simulink model "PendulumQuickStart_RL"  (R2025a)
settings: Solver=ode4  StartTime=0.0  StopTime=inf  FixedStep=0.004  RelTol=1e-3  EnableMultiTasking=on
InitFcn:
  | LoadCalibrateData
  | Linear_System_Model_LQR_Matrixes
values from neighbouring files (symbols this model uses):
  Beq = 30.0    (= 30)    [lqrs13s17_sim.m]
  K = 2/DT    [ol_center_sim.m]
  Kb = 0.11693    [lqrs13s17_sim.m]
  Kt = 0.08505    [lqrs13s17_sim.m]
  Mc = 0.4719    [ol_center_sim.m]
  Mp = 0.1679    [ol_center_sim.m]
  Rm = 2.12    [lqrs13s17_sim.m]
  rmp = 0.013745    [lqrs13s17_sim.m]
undefined symbols (not defined in the file or in its folder): Nbar
libraries: raspberrypiCommlib x2, simulink x1
settings Model: SimulationMode=external  ExtModeTrigDuration=2  Creator=Mustafa  LastModifiedBy=chenyihong
settings SolverCC: ExtrapolationOrder=2.0  AlgebraicLoopSolver=TrustRegion  PositivePriorityOrder=on  AutoInsertRateTranBlk=on
settings DataIOCC: ReturnWorkspaceOutputs=off
settings OptimizationCC: PassReuseOutputArgsAs=Individual arguments  MaxStackSize=200000  EfficientTunableParamExpr=on
settings DebuggingCC: ParameterTunabilityLossMsg=error  UnconnectedInputMsg=warning  UnconnectedOutputMsg=warning  UnconnectedLineMsg=warning  ArithmeticOperatorsInVariantConditions=warning
settings HardwareCC: ProdBitPerLong=64.0  ProdLargestAtomicInteger=LongLong  ProdLargestAtomicFloat=Double  ProdLongLongMode=on  ProdHWDeviceType=ARM Compatible->ARM Cortex-A (64-bit)
settings ModelReferenceCC: EnableRefExpFcnMdlSchedulingChecks=on
settings SFSimCC: SimUseLocalCustomCode=off  CustomCodeUndefinedFunction=UseInterfaceOnly
settings RTWCC: SystemTargetFile=ert.tlc  HardwareBoard=Raspberry Pi (64bit)  TLCOptions="-aInlineSetEventsForThisBaseRateFcn=TLC_FALSE -aSuppressMultiTaskScheduler=TLC_FALSE  -aRateBasedStepFcn=0"  TemplateMakefile=ert_default_tmf  GenerateReport=on  RTWUseLocalCustomCode=off  Toolchain=GNU GCC Embedded Linux  BuildConfiguration=Faster Runs  IncludeHyperlinkInReport=on  LaunchReport=on  GenerateTraceInfo=on  GenerateTraceReport=on  GenerateTraceReportSl=on  GenerateTraceReportSf=on  GenerateTraceReportEml=on  GPUComputeCapability=3.5  DLArmComputeVersion=19.05  Description=Embedded Coder
settings CodeAppCC: ForceParamTrailComments=on  IgnoreCustomStorageClasses=off  OperatorAnnotations=on  SimulinkDataObjDesc=on  SFDataObjDesc=on  InsertBlockDesc=on
settings ERTTargetCC: ExtMode=on  ExtModeTransport=2.0  ExtModeMexArgs='127.0.0.1' 0 17725  InlinedParameterPlacement=Hierarchical  DynamicArrayContainerType=coder::array  CodeReplacementLibrary=ARM Cortex-A CMSIS  SupportContinuousTime=on  SupportVariableSizeSignals=on
settings SimscapeCC: SimscapeLogDecimation=1  SimscapeLogDataHistory=5000

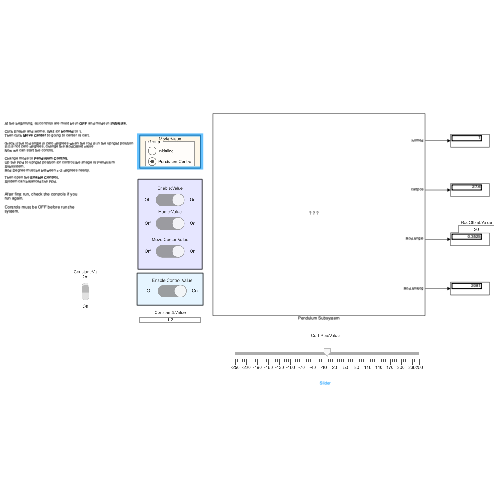
[thumbnail: Simulink's stored preview of the top-level diagram]
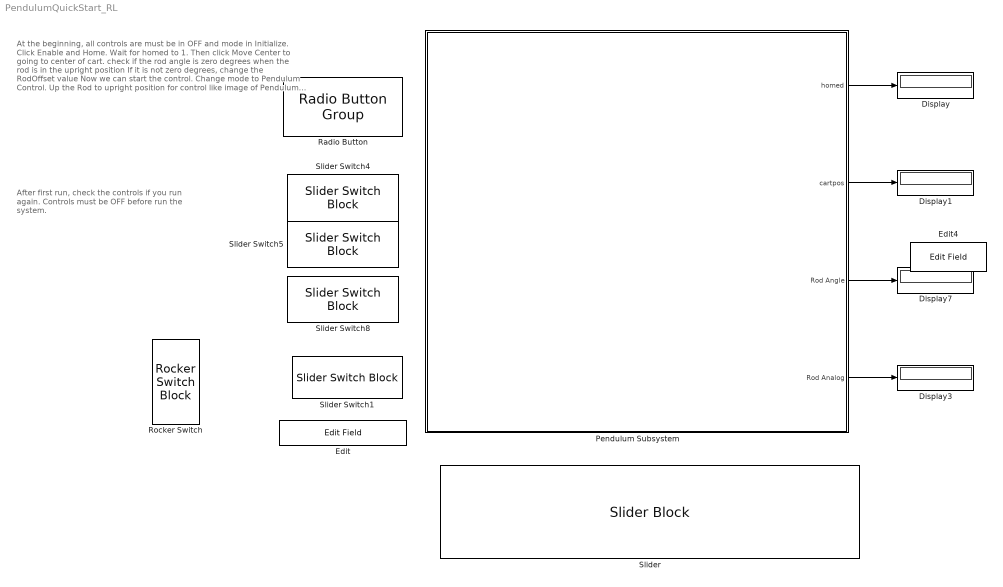
== system PendulumQuickStart_RL ==
  note: At the beginning, all controls are must be in OFF and mode in Initialize.
      |
      | Click Enable and Home. Wait for homed to 1.
      | Then click Move Center to going to center of cart.
      |
      | check if the rod angle is zero degrees when the rod is in the upright position
      | If it is not zero degrees, change the RodOffset value
      | Now we can start the control.
      |
      | Change mode to Pendulum Control.
      | Up the Rod to upright position for control like image of Pendulum Subsystem.
      | Rod Degree must be between +-2 degrees nearly.
      |
      | Then open the Enable Control.
      | System can balanced the Rod.
  note: After first run, check the controls if you run again.
      |
      | Controls must be OFF before run the system.
  Display{,1,3,7} (4 alike) : Display
  Edit : EditField  ShowInitialText=on  Alignment=Center
  Edit4 : EditField  Alignment=Center
  Pendulum Subsystem : Subsystem
      mask Display: image('Resim1.png'); % Use "Edit Image" on toolstrip to change.
  Radio Button : RadioButtonGroup  SelectedLabel=Pendulum Control  ButtonGroupName=Group
  Rocker Switch : RockerSwitchBlock
  Slider : SliderBlock  ScaleMin=-250  ScaleMax=250
  Slider Switch{1,4..5,8} (4 alike) : SliderSwitchBlock
  wires:
  Pendulum Subsystem/1(homed) -> Display/1
  Pendulum Subsystem/2(cartpos) -> Display1/1
  Pendulum Subsystem/3(Rod Angle) -> Display7/1
  Pendulum Subsystem/4(Rod Analog) -> Display3/1

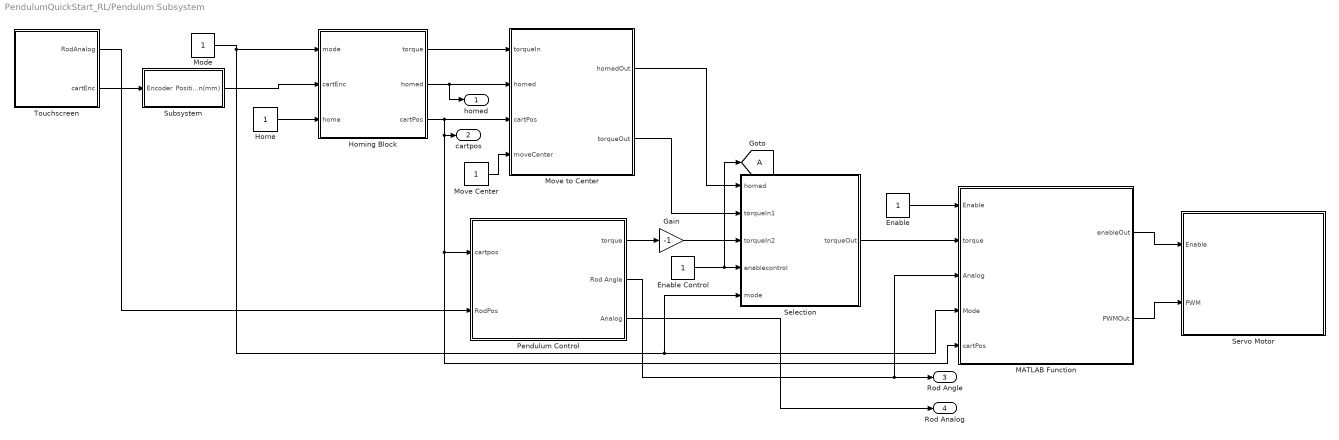
== system PendulumQuickStart_RL/Pendulum Subsystem ==
  Enable : Constant
  Enable Control : Constant
  Gain : Gain  Gain=-1
  Goto : Goto  TagVisibility=global
  Home : Constant
  Homing Block : MATLAB Function  TreatAsAtomicUnit=on
  MATLAB Function : MATLAB Function  TreatAsAtomicUnit=on
  Mode : Constant
  Move Center : Constant
  Move to Center : MATLAB Function  TreatAsAtomicUnit=on
  Pendulum Control : Subsystem
  Selection : MATLAB Function  TreatAsAtomicUnit=on
  Servo Motor : Subsystem
  Subsystem : Subsystem
  Touchscreen : Subsystem
  homed : Outport
  cartpos : Outport  Port=2
  Rod Angle : Outport  Port=3
  Rod Analog : Outport  Port=4
  wires:
  Mode/1 -> Selection/5(mode), MATLAB Function/4(Mode), Homing Block/1(mode)
  Homing Block/2(homed) -> homed/1, Move to Center/2(homed)
  Home/1 -> Homing Block/3(home)
  Move Center/1 -> Move to Center/4(moveCenter)
  Pendulum Control/1(torque) -> Gain/1
  Homing Block/1(torque) -> Move to Center/1(torqueIn)
  Move to Center/1(homedOut) -> Selection/1(homed)
  Move to Center/2(torqueOut) -> Selection/2(torqueIn1)
  Selection/1(torqueOut) -> MATLAB Function/2(torque)
  Enable Control/1 -> Goto/1, Selection/4(enablecontrol)
  MATLAB Function/1(enableOut) -> Servo Motor/1(Enable)
  Pendulum Control/2(Rod Angle) -> MATLAB Function/3(Analog), Rod Angle/1
  Enable/1 -> MATLAB Function/1(Enable)
  Touchscreen/2(cartEnc) -> Subsystem/1(Encoder)
  Subsystem/1(Position(mm)) -> Homing Block/2(cartEnc)
  Pendulum Control/3(Analog) -> Rod Analog/1
  Homing Block/3(cartPos) -> MATLAB Function/5(cartPos), Pendulum Control/1(cartpos), cartpos/1, Move to Center/3(cartPos)
  Touchscreen/1(RodAnalog) -> Pendulum Control/2(RodPos)
  MATLAB Function/2(PWMOut) -> Servo Motor/2(PWM)
  Gain/1 -> Selection/3(torqueIn2)

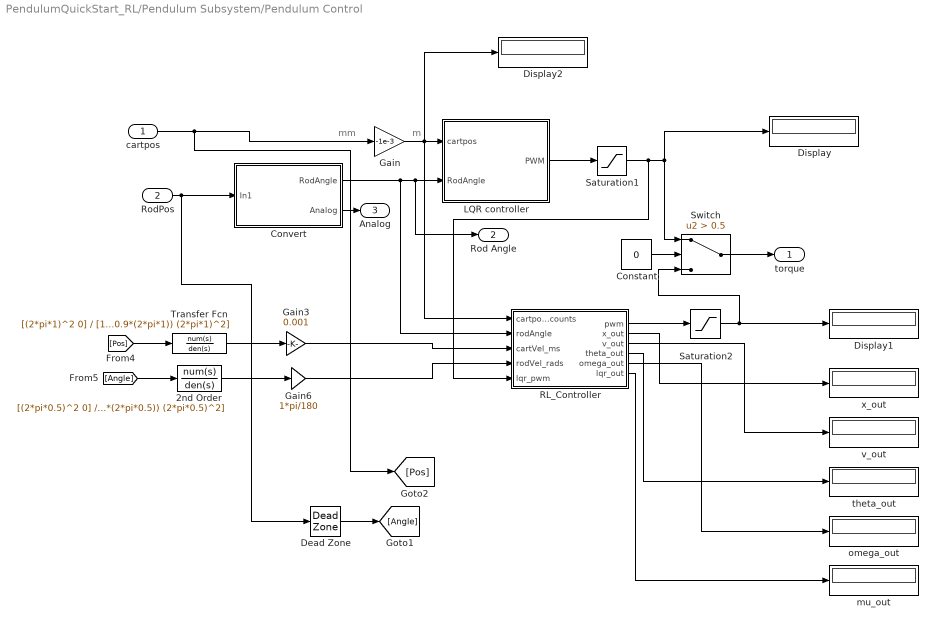
== system PendulumQuickStart_RL/Pendulum Subsystem/Pendulum Control ==
  note: m
  note: mm
  cartpos : Inport
  RodPos : Inport  Port=2
  2nd Order : TransferFcn  Numerator=[(2*pi*0.5)^2 0]  Denominator=[1 (2*0.9*(2*pi*0.5)) (2*pi*0.5)^2]
  Constant : Constant  Value=0
  Convert : Subsystem
  Dead Zone : DeadZone  LowerValue=-0.05  UpperValue=+0.05
  Display : Display
  Display1 : Display
  Display2 : Display
  Gain : Gain  Gain=-1e-3
  Gain3 : Gain  Gain=0.001
  Gain6 : Gain  Gain=1*pi/180
  LQR controller : Subsystem
  RL_Controller : MATLAB Function  TreatAsAtomicUnit=on
  Saturation1 : Saturate  UpperLimit=1000  LowerLimit=-1000
  Saturation2 : Saturate  UpperLimit=1000  LowerLimit=-1000
  Switch : Switch  Criteria=u2 > Threshold  Threshold=0.5  SaturateOnIntegerOverflow=off  InputSameDT=off
  Transfer Fcn : TransferFcn  Numerator=[(2*pi*1)^2 0]  Denominator=[1 (2*0.9*(2*pi*1)) (2*pi*1)^2]
  mu_out : Display
  omega_out : Display
  theta_out : Display
  v_out : Display
  x_out : Display
  torque : Outport
  Rod Angle : Outport  Port=2
  Analog : Outport  Port=3
  wires:
  cartpos/1 -> Gain/1, [Pos]
  Convert/2(Analog) -> Analog/1
  RodPos/1 -> Dead Zone/1, Convert/1(In1)
  Transfer Fcn/1 -> Gain3/1
  2nd Order/1 -> Gain6/1
  [Pos] -> Transfer Fcn/1
  [Angle] -> 2nd Order/1
  Saturation1/1 -> RL_Controller/5(lqr_pwm), Switch/1, Display/1
  Constant/1 -> Switch/2
  Switch/1 -> torque/1
  Dead Zone/1 -> [Angle]
  LQR controller/1(PWM) -> Saturation1/1
  Gain6/1 -> RL_Controller/4(rodVel_rads)
  RL_Controller/1(pwm) -> Saturation2/1
  Saturation2/1 -> Switch/3, Display1/1
  Gain/1 -> Display2/1, RL_Controller/1(cartpos_counts), LQR controller/1(cartpos)
  Convert/1(RodAngle) -> RL_Controller/2(rodAngle), LQR controller/2(RodAngle), Rod Angle/1
  Gain3/1 -> RL_Controller/3(cartVel_ms)
  RL_Controller/2(x_out) -> x_out/1
  RL_Controller/3(v_out) -> v_out/1
  RL_Controller/4(theta_out) -> theta_out/1
  RL_Controller/5(omega_out) -> omega_out/1
  RL_Controller/6(lqr_out) -> mu_out/1

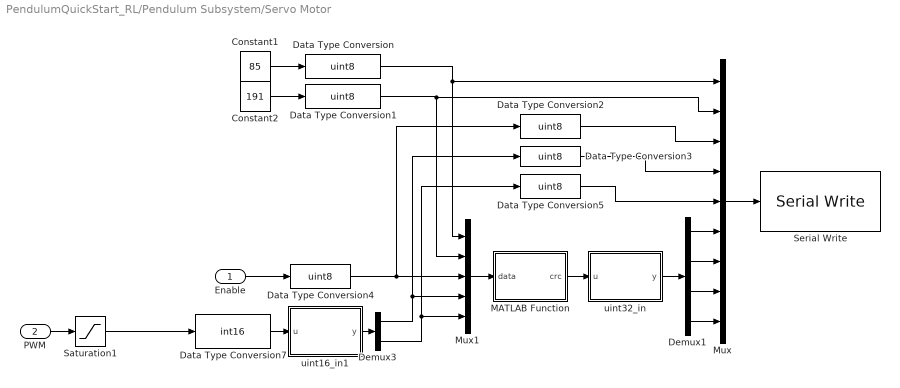
== system PendulumQuickStart_RL/Pendulum Subsystem/Servo Motor ==
  Enable : Inport
  PWM : Inport  Port=2
  Constant1 : Constant  Value=85
  Constant2 : Constant  Value=191
  Data Type Conversion{,1..5} (6 alike) : DataTypeConversion  OutDataTypeStr=uint8  SaturateOnIntegerOverflow=off  RndMeth=Floor
  Data Type Conversion7 : DataTypeConversion  OutDataTypeStr=int16  SaturateOnIntegerOverflow=off  RndMeth=Floor
  Demux1 : Demux
  Demux3 : Demux  Outputs=2
  MATLAB Function : MATLAB Function  TreatAsAtomicUnit=on
  Mux : Mux  Inputs=9
  Mux1 : Mux  Inputs=5
  Saturation1 : Saturate  UpperLimit=1000  LowerLimit=-1000
  Serial Write : raspberrypiCommlib/Serial Write  board=Pi 3 Model B  SCIModule_=/dev/serial0  Baudrate_=115200  Parity=None  StopBits_=1  HardwareFlowControl=None  ByteOrder=LittleEndian  OutputStatus=off  blockPlatform=RaspberryPi
  uint16_in1 : MATLAB Function  TreatAsAtomicUnit=on
  uint32_in : MATLAB Function  TreatAsAtomicUnit=on
  wires:
  Data Type Conversion7/1 -> uint16_in1/1(u)
  uint16_in1/1(y) -> Demux3/1
  Data Type Conversion5/1 -> Mux/5
  Demux3/1 -> Data Type Conversion3/1, Mux1/4
  Data Type Conversion/1 -> Mux/1, Mux1/1
  Data Type Conversion3/1 -> Mux/4
  Data Type Conversion1/1 -> Mux/2, Mux1/2
  Mux/1 -> Serial Write/1
  Data Type Conversion2/1 -> Mux/3
  uint32_in/1(y) -> Demux1/1
  MATLAB Function/1(crc) -> uint32_in/1(u)
  Mux1/1 -> MATLAB Function/1(data)
  Enable/1 -> Data Type Conversion4/1
  Constant2/1 -> Data Type Conversion1/1
  Constant1/1 -> Data Type Conversion/1
  Demux3/2 -> Data Type Conversion5/1, Mux1/5
  Demux1/4 -> Mux/9
  Demux1/3 -> Mux/8
  Demux1/2 -> Mux/7
  Demux1/1 -> Mux/6
  Data Type Conversion4/1 -> Mux1/3, Data Type Conversion2/1
  PWM/1 -> Saturation1/1
  Saturation1/1 -> Data Type Conversion7/1

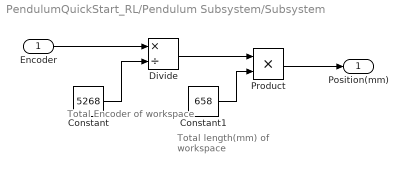
== system PendulumQuickStart_RL/Pendulum Subsystem/Subsystem ==
  note: Total length(mm)
      | of workspace
  note: Total Encoder
      | of workspace
  Encoder : Inport
  Constant : Constant  Value=5268
  Constant1 : Constant  Value=658
  Divide : Product  Inputs=*/
  Product : Product
  Position(mm) : Outport  VectorParamsAs1DForOutWhenUnconnected=off
  wires:
  Encoder/1 -> Divide/1
  Constant1/1 -> Product/2
  Divide/1 -> Product/1
  Constant/1 -> Divide/2
  Product/1 -> Position(mm)/1

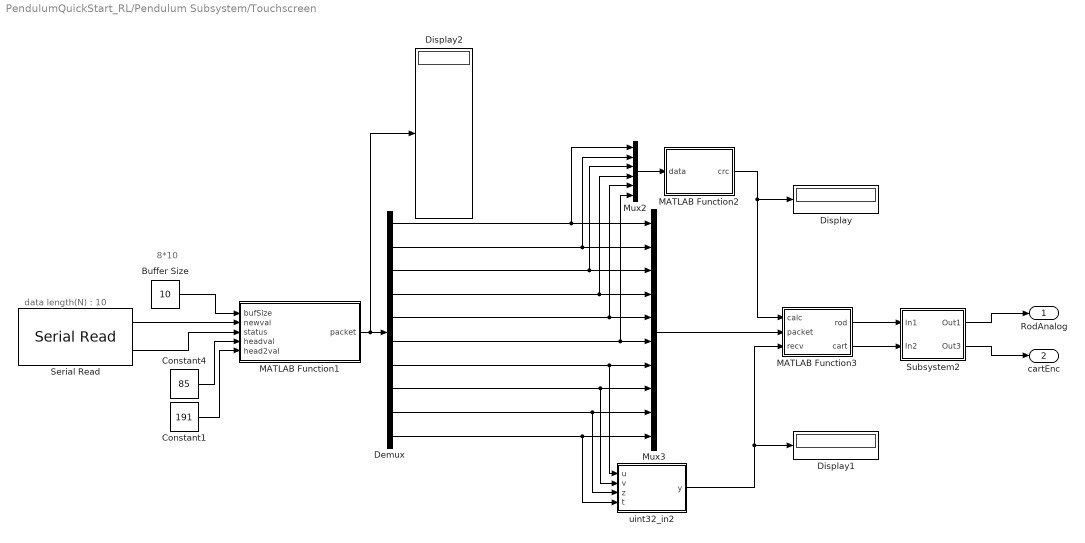
== system PendulumQuickStart_RL/Pendulum Subsystem/Touchscreen ==
  note: data length(N) : 10
  note: 8*10
  Buffer Size : Constant  Value=10  OutDataTypeStr=uint8
  Constant1 : Constant  Value=191  OutDataTypeStr=uint8
  Constant4 : Constant  Value=85  OutDataTypeStr=uint8
  Demux : Demux  Outputs=10
  Display : Display
  Display1 : Display
  Display2 : Display
  MATLAB Function1 : MATLAB Function  TreatAsAtomicUnit=on
  MATLAB Function2 : MATLAB Function  TreatAsAtomicUnit=on
  MATLAB Function3 : MATLAB Function  TreatAsAtomicUnit=on
  Mux2 : Mux  Inputs=6
  Mux3 : Mux  Inputs=10
  Serial Read : raspberrypiCommlib/Serial Read  board=Pi 3 Model B  SCIModule_=/dev/serial0  Baudrate_=115200  Parity=None  StopBits_=1  HardwareFlowControl=None  ByteOrder=LittleEndian  DataLength=10  DataType=uint8  OutputStatus=on  SampleTime=0.004  blockPlatform=RaspberryPi
  Subsystem2 : Subsystem
  uint32_in2 : MATLAB Function  TreatAsAtomicUnit=on
  RodAnalog : Outport
  cartEnc : Outport  Port=2
  wires:
  Demux/1 -> Mux3/1, Mux2/1
  Demux/6 -> Mux3/6, Mux2/6
  Subsystem2/1(Out1) -> RodAnalog/1
  Mux2/1 -> MATLAB Function2/1(data)
  Constant1/1 -> MATLAB Function1/5(head2val)
  MATLAB Function3/2(cart) -> Subsystem2/2(In2)
  Demux/4 -> Mux3/4, Mux2/4
  Demux/10 -> Mux3/10, uint32_in2/4(t)
  Demux/3 -> Mux3/3, Mux2/3
  uint32_in2/1(y) -> Display1/1, MATLAB Function3/3(recv)
  Demux/8 -> Mux3/8, uint32_in2/2(v)
  Buffer Size/1 -> MATLAB Function1/1(bufSize)
  Demux/5 -> Mux3/5, Mux2/5
  Demux/2 -> Mux3/2, Mux2/2
  Constant4/1 -> MATLAB Function1/4(headval)
  Serial Read/2 -> MATLAB Function1/3(status)
  Mux3/1 -> MATLAB Function3/2(packet)
  MATLAB Function2/1(crc) -> Display/1, MATLAB Function3/1(calc)
  MATLAB Function1/1(packet) -> Display2/1, Demux/1
  Demux/7 -> Mux3/7, uint32_in2/1(u)
  Subsystem2/2(Out3) -> cartEnc/1
  MATLAB Function3/1(rod) -> Subsystem2/1(In1)
  Demux/9 -> Mux3/9, uint32_in2/3(z)
  Serial Read/1 -> MATLAB Function1/2(newval)

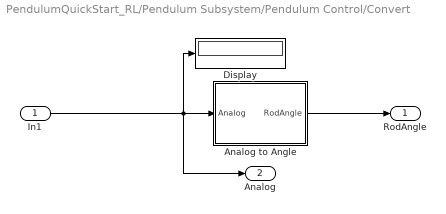
== system PendulumQuickStart_RL/Pendulum Subsystem/Pendulum Control/Convert ==
  In1 : Inport
  Analog to Angle : Subsystem
  Display : Display
  RodAngle : Outport
  Analog : Outport  Port=2
  wires:
  In1/1 -> Analog/1, Display/1, Analog to Angle/1(Analog)
  Analog to Angle/1(RodAngle) -> RodAngle/1

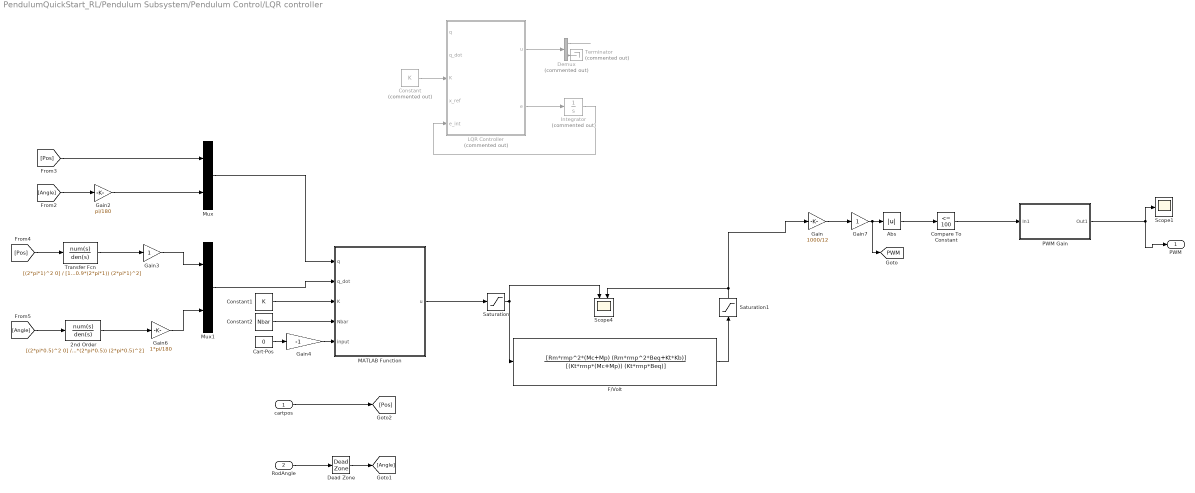
== system PendulumQuickStart_RL/Pendulum Subsystem/Pendulum Control/LQR controller ==
  cartpos : Inport
  RodAngle : Inport  Port=2
  2nd Order : TransferFcn  Numerator=[(2*pi*0.5)^2 0]  Denominator=[1 (2*0.9*(2*pi*0.5)) (2*pi*0.5)^2]
  Abs : Abs  SaturateOnIntegerOverflow=off
  Cart-Pos : Constant  Value=0
  Compare To Constant : simulink/Logic and Bit Operations/Compare To Constant  relop=<=  const=100  OutDataTypeStr=boolean
  Constant : Constant  Commented=on  Value=K  VectorParams1D=off
  Constant1 : Constant  Value=K  VectorParams1D=off
  Constant2 : Constant  Value=Nbar  VectorParams1D=off
  Dead Zone : DeadZone  LowerValue=-0.05  UpperValue=+0.05
  Demux : Demux  Commented=on  Outputs=2
  F/Volt : TransferFcn  Numerator=[Rm*rmp^2*(Mc+Mp) (Rm*rmp^2*Beq+Kt*Kb)]  Denominator=[(Kt*rmp*(Mc+Mp)) (Kt*rmp*Beq)]
  Gain : Gain  Gain=1000/12
  Gain2 : Gain  Gain=pi/180
  Gain3 : Gain
  Gain4 : Gain  Gain=-1
  Gain6 : Gain  Gain=1*pi/180
  Gain7 : Gain
  Integrator : Integrator  Commented=on
  LQR Controller : MATLAB Function  Commented=on  TreatAsAtomicUnit=on
  MATLAB Function : MATLAB Function  TreatAsAtomicUnit=on
  Mux : Mux  Inputs=2
  Mux1 : Mux  Inputs=2
  PWM Gain : Subsystem
      mask Display: image('Screenshot 2024-12-13 121633.png');
  Saturation : Saturate  UpperLimit=35  LowerLimit=-35
  Saturation1 : Saturate  UpperLimit=1000  LowerLimit=-1000
  Scope1 : Scope
      settings: ActiveDisplayYMinimum=895.90874  ActiveDisplayYMaximum=1929.7569
  Scope4 : Scope  NumInputPorts=2
      settings: TimeSpan=240  ActiveDisplayYMinimum=-43.75  ActiveDisplayYMaximum=43.75  DataLoggingVariableName=ScopeData2
  Terminator : Terminator  Commented=on
  Transfer Fcn : TransferFcn  Numerator=[(2*pi*1)^2 0]  Denominator=[1 (2*0.9*(2*pi*1)) (2*pi*1)^2]
  PWM : Outport
  tag scope: PWM=global
  wires:
  Constant/1 -> LQR Controller/3(K)
  LQR Controller/2(e) -> Integrator/1
  ? -> LQR Controller/1(q)
  LQR Controller/1(u) -> Demux/1
  Integrator/1 -> LQR Controller/5(e_int)
  ? -> LQR Controller/2(q_dot)
  Demux/1 -> ?
  ? -> LQR Controller/4(x_ref)
  Demux/2 -> Terminator/1
  Gain2/1 -> Mux/2
  Gain6/1 -> Mux1/2
  Gain/1 -> Gain7/1
  RodAngle/1 -> Dead Zone/1
  Constant1/1 -> MATLAB Function/3(K)
  Mux1/1 -> MATLAB Function/2(q_dot)
  MATLAB Function/1(u) -> Saturation/1
  Cart-Pos/1 -> Gain4/1
  Mux/1 -> MATLAB Function/1(q)
  Constant2/1 -> MATLAB Function/4(Nbar)
  F/Volt/1 -> Saturation1/1
  Gain7/1 -> [PWM], Abs/1
  Saturation1/1 -> Gain/1, Scope4/2
  Saturation/1 -> F/Volt/1, Scope4/1
  2nd Order/1 -> Gain6/1
  Transfer Fcn/1 -> Gain3/1
  Gain3/1 -> Mux1/1
  Abs/1 -> Compare To Constant/1
  Gain4/1 -> MATLAB Function/5(input)
  Dead Zone/1 -> [Angle]
  cartpos/1 -> [Pos]
  [Angle] -> Gain2/1
  [Pos] -> Mux/1
  [Pos] -> Transfer Fcn/1
  [Angle] -> 2nd Order/1
  PWM Gain/1(Out1) -> PWM/1, Scope1/1
  Compare To Constant/1 -> PWM Gain/1(In1)

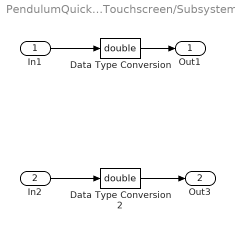
== system PendulumQuickStart_RL/Pendulum Subsystem/Touchscreen/Subsystem2 ==
  In1 : Inport
  In2 : Inport  Port=2
  Data Type Conversion : DataTypeConversion  OutDataTypeStr=double  SaturateOnIntegerOverflow=off  RndMeth=Floor
  Data Type Conversion2 : DataTypeConversion  OutDataTypeStr=double  SaturateOnIntegerOverflow=off  RndMeth=Floor
  Out1 : Outport
  Out3 : Outport  Port=2
  wires:
  Data Type Conversion2/1 -> Out3/1
  Data Type Conversion/1 -> Out1/1
  In2/1 -> Data Type Conversion2/1
  In1/1 -> Data Type Conversion/1

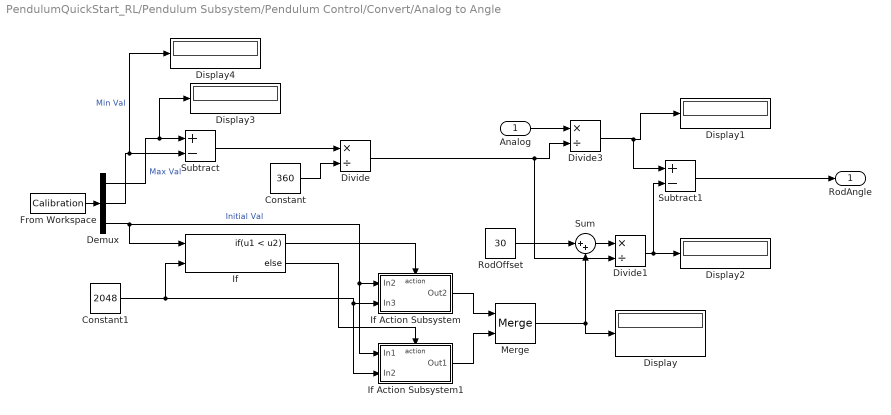
== system PendulumQuickStart_RL/Pendulum Subsystem/Pendulum Control/Convert/Analog to Angle ==
  Analog : Inport
  Constant : Constant  Value=360
  Constant1 : Constant  Value=2048
  Demux : Demux  Outputs=3
  Display{,1..4} (5 alike) : Display
  Divide : Product  Inputs=*/
  Divide1 : Product  Inputs=*/
  Divide3 : Product  Inputs=*/
  From Workspace : FromWorkspace  VariableName=Calibration
  If : If  NumInputs=2  IfExpression=u1 < u2
  If Action Subsystem : Subsystem  TreatAsAtomicUnit=on
  If Action Subsystem1 : Subsystem  TreatAsAtomicUnit=on
  Merge : Merge
  RodOffset : Constant  Value=30
  Subtract : Sum  Inputs=+-
  Subtract1 : Sum  Inputs=+-
  Sum : Sum  Inputs=|++
  RodAngle : Outport
  wires:
  From Workspace/1 -> Demux/1
  Demux/3 -> If/1, If Action Subsystem/1(In2), If Action Subsystem1/1(In1)  "Initial Val"
  Constant1/1 -> If/2, If Action Subsystem/2(In3), If Action Subsystem1/2(In2)
  If/1 -> If Action Subsystem/Action
  If/2 -> If Action Subsystem1/Action
  If Action Subsystem1/1(Out1) -> Merge/2
  If Action Subsystem/1(Out2) -> Merge/1
  Merge/1 -> Sum/2, Display/1
  Demux/1 -> Display3/1, Subtract/1  "Max Val"
  Demux/2 -> Display4/1, Subtract/2  "Min Val"
  Constant/1 -> Divide/2
  Subtract/1 -> Divide/1
  Divide/1 -> Divide1/2, Divide3/2
  Analog/1 -> Divide3/1
  Divide1/1 -> Display2/1, Subtract1/2
  Divide3/1 -> Display1/1, Subtract1/1
  RodOffset/1 -> Sum/1
  Sum/1 -> Divide1/1
  Subtract1/1 -> RodAngle/1

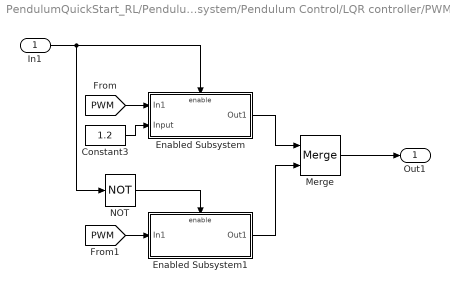
== system PendulumQuickStart_RL/Pendulum Subsystem/Pendulum Control/LQR controller/PWM Gain ==
  In1 : Inport
  Constant3 : Constant  Value=1.2
  Enabled Subsystem : Subsystem  TreatAsAtomicUnit=on
  Enabled Subsystem1 : Subsystem  TreatAsAtomicUnit=on
  Merge : Merge
  NOT : Logic  Operator=NOT  IconShape=distinctive  AllPortsSameDT=off  OutDataTypeStr=boolean
  Out1 : Outport
  wires:
  [PWM] -> Enabled Subsystem/1(In1)
  In1/1 -> NOT/1, Enabled Subsystem/Enable
  Constant3/1 -> Enabled Subsystem/2(Input)
  Enabled Subsystem1/1(Out1) -> Merge/2
  [PWM] -> Enabled Subsystem1/1(In1)
  NOT/1 -> Enabled Subsystem1/Enable
  Enabled Subsystem/1(Out1) -> Merge/1
  Merge/1 -> Out1/1

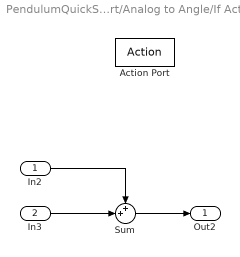
== system PendulumQuickStart_RL/Pendulum Subsystem/Pendulum Control/Convert/Analog to Angle/If Action Subsystem ==
  In2 : Inport
  In3 : Inport  Port=2
  Action Port : ActionPort  ActionPortLabel=if(u1 < u2)
  Sum : Sum  Inputs=++|
  Out2 : Outport  VectorParamsAs1DForOutWhenUnconnected=off
  wires:
  In2/1 -> Sum/1
  Sum/1 -> Out2/1
  In3/1 -> Sum/2

== system PendulumQuickStart_RL/Pendulum Subsystem/Pendulum Control/Convert/Analog to Angle/If Action Subsystem1 ==
  In1 : Inport
  In2 : Inport  Port=2
  Action Port : ActionPort  ActionPortLabel=else
  Sum : Sum  Inputs=+-|
  Out1 : Outport  VectorParamsAs1DForOutWhenUnconnected=off
  wires:
  In1/1 -> Sum/1
  In2/1 -> Sum/2
  Sum/1 -> Out1/1

== system PendulumQuickStart_RL/Pendulum Subsystem/Pendulum Control/LQR controller/PWM Gain/Enabled Subsystem ==
  In1 : Inport
  Input : Inport  Port=2
  Enable : EnablePort
  Product : Product
  Out1 : Outport
  wires:
  In1/1 -> Product/1
  Input/1 -> Product/2
  Product/1 -> Out1/1

== system PendulumQuickStart_RL/Pendulum Subsystem/Pendulum Control/LQR controller/PWM Gain/Enabled Subsystem1 ==
  In1 : Inport
  Enable : EnablePort
  Out1 : Outport
  wires:
  In1/1 -> Out1/1

== matlab function PendulumQuickStart_RL/Pendulum Subsystem/Selection ==
  settings: updateMethod=DISCRETE
  data: homed input; torqueIn1 input; torqueOut output; torqueIn2 input; enablecontrol input; mode input
function torqueOut  =fcn(homed,torqueIn1,torqueIn2,enablecontrol,mode)
persistent torqueval

if isempty(torqueval)
    torqueval=0;
end

if (mode==0)
    torqueval=torqueIn1;
end
if (mode==1)
    if (homed==1)
        if (enablecontrol==1)
            torqueval=torqueIn2;
        else
            torqueval=0;
        end
    end
end

torqueOut=torqueval;
end

== matlab function PendulumQuickStart_RL/Pendulum Subsystem/Servo Motor/MATLAB Function ==
  data: data input; crc output
function crc = crc_32(data)

% Computes the CRC-32/MPEG-2 checksum value of a byte vector.
% Uses a left shifting (not reflected) CRC along with the 
% CRC polynomial 0x04C11DB7 and initial CRC value of 0xFFFFFFFF,
% and is not post complemented.
%--------------------------------------------------------------------------
%   Version:    130
%   Programmer: Oliver Calderbank
%   Date:       21-07-2019

% Initialize variables
crc  = uint32(hex2dec('FFFFFFFF'));
poly = uint32(hex2dec('04C11DB7'));
data = uint8(data);
temp = uint32(data);

for i = 1:length(data)
    % xor next byte to upper bits of crc
    crc = bitxor(crc,uint32(bitshift(temp(i),24)));
    for j = 1:8
        msb = bitsra(crc,31);
        crc = bitsll(crc,1);
        if msb == 1 
            crc = bitxor(crc,poly);
        end 
    end
end
end

== matlab function PendulumQuickStart_RL/Pendulum Subsystem/Pendulum Control/RL_Controller ==
  settings: updateMethod=DISCRETE
  data: cartpos_counts input; pwm output; rodAngle input; cartVel_ms input; rodVel_rads input; x_out output; v_out output; theta_out output; omega_out output; lqr_out output; lqr_pwm input
function [pwm, x_out, v_out, theta_out, omega_out, lqr_out] = fcn_LQR_static(cartpos_counts, rodAngle, cartVel_ms, rodVel_rads, lqr_pwm)
%#codegen
% =========================================================================
% 原厂 LQR 干净静置（上机用）。贴进 RL_Controller 的 MATLAB Function 块时，只把第一行的函数名改回 fcn。
% 接口与 fcn_LQR_probe150.m 相同（5 个输入，第 5 个 lqr_pwm 接原厂 LQR 的输出），不用改线。
% 控制完全由原厂 LQR 块负责，本函数原样转发，不加探测、不加脉冲。
% 目的：10/02 只有 18 s 静置且小车在漂，模型 v1 的静置部分对原厂 LQR 准不准没法判（预测 2.5°，实测 1.6°）。
% 扶正后静置至少 150 s，不碰。第 6 路输出 lqr_out = 原厂 LQR 的 PWM。
% =========================================================================
V_SIGN      = -1.0;       % 勿改（只用于记录）
OMEGA_SCALE = 360/2048;

pwm = lqr_pwm;
if pwm >  1000.0, pwm =  1000.0; end
if pwm < -1000.0, pwm = -1000.0; end

x_out = cartpos_counts; v_out = V_SIGN * cartVel_ms; theta_out = rodAngle * (pi / 180);
omega_out = OMEGA_SCALE * rodVel_rads; lqr_out = lqr_pwm;
end

== matlab function PendulumQuickStart_RL/Pendulum Subsystem/Servo Motor/uint16_in1 ==
  data: u input; y output
function y = fcn(u)
t=typecast(int16(u),'uint8');
y = [t(1) t(2)];

== matlab function PendulumQuickStart_RL/Pendulum Subsystem/Touchscreen/uint32_in2 ==
  data: u input; y output uint32 size=1; v input; z input; t input
function y = fcn(u,v,z,t)
x=[u v z t];
k=typecast(uint8(x),'uint32');
y = k;

== matlab function PendulumQuickStart_RL/Pendulum Subsystem/MATLAB Function ==
  data: Enable input; torque input; Analog input; Mode input; enableOut output; PWMOut output; cartPos input
function [enableOut,PWMOut] = fcn(Enable,torque,Analog,Mode,cartPos)
    if (Enable==1)
        enableOut=1;
        if (Mode==0)
            PWMOut=torque;
        else
            if ((abs(Analog)<= 30) && (abs(cartPos)<= 340))
                PWMOut=torque;
            else
                enableOut=0;
                PWMOut=0;
            end
        end
    else
        enableOut=0;
        PWMOut=0;
    end
end

== matlab function PendulumQuickStart_RL/Pendulum Subsystem/Pendulum Control/LQR controller/LQR Controller ==
  data: q input; u output; q_dot input; K input; x_ref input; e_int input; e output
function [u,e] = fcn(q,q_dot,K,x_ref,e_int)

%%States
x = q(1,1);
theta = q(2,1);
x_dot = q_dot(1,1);
theta_dot = q_dot(2,1);

LQR_states = [x;
              theta;
              x_dot;
              theta_dot;
              e_int];
u_int = K*LQR_states;

u = [u_int;
     0];
e= x - x_ref;

end

== matlab function PendulumQuickStart_RL/Pendulum Subsystem/Touchscreen/MATLAB Function3 ==
  data: calc input; packet input; rod output int16 size=1; recv input; cart output int16 size=1
function [rod,cart] = fcn(calc,packet,recv)
persistent validpack;
persistent validpack2;
if isempty(validpack)
    Axisx=[packet(3) packet(4)];
    validpack=typecast(uint8(Axisx),'int16');
end
if isempty(validpack2)
    Axisy=[packet(5) packet(6)];
    validpack2=typecast(uint8(Axisy),'int16');
end
if calc==recv
    Axisx=[packet(3) packet(4)];
    validpack=typecast(uint8(Axisx),'int16');
    Axisy=[packet(5) packet(6)];
    validpack2=typecast(uint8(Axisy),'int16');
    rod=validpack;
    cart=validpack2;
else
	rod=validpack;
    cart=validpack2;
end

== matlab function PendulumQuickStart_RL/Pendulum Subsystem/Touchscreen/MATLAB Function2 ==
  data: data input; crc output
function crc = crc_32(data)

% Computes the CRC-32/MPEG-2 checksum value of a byte vector.
% Uses a left shifting (not reflected) CRC along with the 
% CRC polynomial 0x04C11DB7 and initial CRC value of 0xFFFFFFFF,
% and is not post complemented.
%--------------------------------------------------------------------------
%   Version:    130
%   Programmer: Oliver Calderbank
%   Date:       21-07-2019

% Initialize variables
crc  = uint32(hex2dec('FFFFFFFF'));
poly = uint32(hex2dec('04C11DB7'));
data = uint8(data);
temp = uint32(data);

for i = 1:length(data)
    % xor next byte to upper bits of crc
    crc = bitxor(crc,uint32(bitshift(temp(i),24)));
    for j = 1:8
        msb = bitsra(crc,31);
        crc = bitsll(crc,1);
        if msb == 1 
            crc = bitxor(crc,poly);
        end 
    end
end
end

== matlab function PendulumQuickStart_RL/Pendulum Subsystem/Pendulum Control/LQR controller/MATLAB Function ==
  data: q input; u output; q_dot input; K input; Nbar input; input input
function u = fcn(q,q_dot,K,Nbar,input)
input = Nbar*input*1e-3;

%%States
x = q(1,1);
theta = q(2,1);
x_dot = q_dot(1,1);
theta_dot = q_dot(2,1);

LQR_states = [x;
              theta;
              x_dot;
              theta_dot];

u=input-K*LQR_states

end

== matlab function PendulumQuickStart_RL/Pendulum Subsystem/Homing Block ==
  settings: updateMethod=DISCRETE
  data: torque output; mode input; cartEnc input; home input; homed output; cartPos output
function [torque,homed,cartPos]=fcn(mode,cartEnc,home)
persistent torqueval
persistent state
persistent precartEnc
persistent homeval
persistent counter
persistent i
persistent precart
persistent prepos
persistent precartArray

if isempty(state)
    torqueval=0;
    state=0;
    precartEnc=0;
    precartArray=[0 0 0 0 0 0 0 0 0 0];
    homeval=0;
    counter=0;
    i=0;
    precart=0;
    prepos=0;
end

if (mode==0)
    if (homeval==0)
        if (home==0)
            state=0;
            homeval=0;
            counter=0;
            precart=0;
            prepos=0;
            precartArray=[0 0 0 0 0 0 0 0 0 0];
        end
        if (state==0)
            torqueval=0;
            if (home==1)
                state=1;
            end
        elseif (state==1)
            torqueval=-550;
            state=2;
        elseif (state==2) % 4 sec wait and check final cartpos
            if (counter==150)
                if (all(precartArray==cartEnc))
                    torqueval=0;
                    homeval=1;
                    prepos=cartEnc;
                else
                      i=i+1;
                      precartArray(i)=precart;
                      if (i==10)
                          i=0;
                      end             
                      precart=cartEnc;
                end
            else
                counter=counter+1;
            end
        end
    else
        if (home==0)
            state=0;
            homeval=0;
            counter=0;
            precartEnc=0;
            prepos=0;
        end
    end
end
homed=homeval;
torque=torqueval;
if (homed==1)
    precartEnc=-329+prepos;
    cartPos=precartEnc-cartEnc;
else
    cartPos=cartEnc;
end
end

== matlab function PendulumQuickStart_RL/Pendulum Subsystem/Servo Motor/uint32_in ==
  data: u input; y output
function y = fcn(u)
t=typecast(uint32(u),'uint8');
y = [t(1) t(2) t(3) t(4)];

== matlab function PendulumQuickStart_RL/Pendulum Subsystem/Touchscreen/MATLAB Function1 ==
  settings: updateMethod=DISCRETE
  data: bufSize input uint8 size=1; newval input uint8 size=10; status input; headval input uint8; packet output size=10; head2val input
function packet   = fcn(bufSize,newval,status,headval,head2val)
%initializing
persistent val;
persistent bff;
persistent packetindex
if isempty(bff)
    packetindex =uint8(zeros(1,10));
end
if isempty(val)
    val=0;
    bff = zeros(bufSize,1); %initializing
    inc=0;
else
    inc=1;
end

ind =uint8( mod(val-1,bufSize) + 1); %current index
if isempty(bff)
    bff = zeros(bufSize,1); %initializing
end
if status==0  %UART Status
    for i = 1:1:10
        bff(mod(ind-1+i-1,bufSize)+1) = newval(i); %adding the circular buffer
    end
    if inc==1
        val=val+10;   
    end
end
if ind==0
    val=0;
end
buffout =uint8( bff((1:80)));  % whole buffer
head=uint8(find(bff(ind+1:end)==headval)+double(ind)); %finding first header
if isempty(head)
    head=uint8(find(bff(1:end)==headval));
end
if bff(mod(head(1),bufSize)+1)==head2val %header2 check
    packetindex=[mod(head(1)-1,bufSize)+1 mod(head(1),bufSize)+1 mod(head(1)+1,bufSize)+1 mod(head(1)+2,bufSize)+1 ... %adding correct package's index to array
                 mod(head(1)+3,bufSize)+1 mod(head(1)+4,bufSize)+1 mod(head(1)+5,bufSize)+1 mod(head(1)+6,bufSize)+1 mod(head(1)+7,bufSize)+1 mod(head(1)+8,bufSize)+1];
end
lastadd=uint8(bff(head(1)+1));
packet=bff(packetindex);

== matlab function PendulumQuickStart_RL/Pendulum Subsystem/Move to Center ==
  data: homedOut output; torqueIn input; torqueOut output; homed input; cartPos input; moveCenter input
function [homedOut, torqueOut] = fcn(torqueIn, homed, cartPos, moveCenter)
%initializing
persistent kp;
persistent set_pos;
if isempty(kp)
    set_pos=0;
    kp=4;
end
if (homed == 1 && moveCenter==1)
   torqueOut=(kp*(set_pos-cartPos));
   if (abs(set_pos-cartPos)<1)
       torqueOut=0;
   end
else
    torqueOut=torqueIn;
end
homedOut=homed;
end
